simulink model "AXU5EV_Encoder_Components"  (R2026b)
settings: Solver=VariableStepAuto
settings Model: Creator=lww  LastModifiedBy=lww

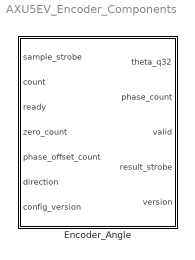
== system AXU5EV_Encoder_Components ==
  Encoder_Angle : Subsystem

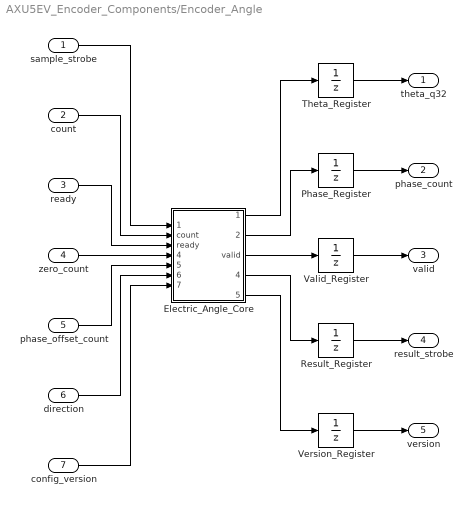
== system AXU5EV_Encoder_Components/Encoder_Angle ==
  sample_strobe : Inport  OutDataTypeStr=boolean  SampleTime=2e-8
  count : Inport  Port=2  OutDataTypeStr=uint32  SampleTime=2e-8
  ready : Inport  Port=3  OutDataTypeStr=boolean  SampleTime=2e-8
  zero_count : Inport  Port=4  OutDataTypeStr=uint32  SampleTime=2e-8
  phase_offset_count : Inport  Port=5  OutDataTypeStr=uint16  SampleTime=2e-8
  direction : Inport  Port=6  OutDataTypeStr=boolean  SampleTime=2e-8
  config_version : Inport  Port=7  OutDataTypeStr=uint32  SampleTime=2e-8
  Electric_Angle_Core : MATLAB Function  TreatAsAtomicUnit=on
  Phase_Register : UnitDelay  SampleTime=2e-8
  Result_Register : UnitDelay  SampleTime=2e-8
  Theta_Register : UnitDelay  SampleTime=2e-8
  Valid_Register : UnitDelay  SampleTime=2e-8
  Version_Register : UnitDelay  SampleTime=2e-8
  theta_q32 : Outport
  phase_count : Outport  Port=2
  valid : Outport  Port=3
  result_strobe : Outport  Port=4
  version : Outport  Port=5
  wires:
  Version_Register/1 -> version/1
  Result_Register/1 -> result_strobe/1
  Valid_Register/1 -> valid/1
  Phase_Register/1 -> phase_count/1
  Theta_Register/1 -> theta_q32/1
  Electric_Angle_Core/1(theta_q32) -> Theta_Register/1
  sample_strobe/1 -> Electric_Angle_Core/1(sample_strobe)
  count/1 -> Electric_Angle_Core/2(count)
  ready/1 -> Electric_Angle_Core/3(ready)
  zero_count/1 -> Electric_Angle_Core/4(zero_count)
  phase_offset_count/1 -> Electric_Angle_Core/5(phase_offset_count)
  direction/1 -> Electric_Angle_Core/6(direction)
  config_version/1 -> Electric_Angle_Core/7(config_version)
  Electric_Angle_Core/2(phase_count) -> Phase_Register/1
  Electric_Angle_Core/3(valid) -> Valid_Register/1
  Electric_Angle_Core/4(result_strobe) -> Result_Register/1
  Electric_Angle_Core/5(version) -> Version_Register/1

== matlab function AXU5EV_Encoder_Components/Encoder_Angle/Electric_Angle_Core ==
  data: sample_strobe input; theta_q32 output; count input; ready input; zero_count input; phase_offset_count input; direction input; config_version input; phase_count output; valid output; result_strobe output; version output
function [theta_q32,phase_count,valid,result_strobe,version] = f(sample_strobe,count,ready,zero_count,phase_offset_count,direction,config_version)
%#codegen
[theta_q32,phase_count,valid,result_strobe,version]=encoder_angle_step(sample_strobe,count,ready,zero_count,phase_offset_count,direction,config_version);
end
